simulink model "project"  (R2022a)
settings: Solver=ode45  StartTime=0.0  StopTime=100  RelTol=1e-3  EnableMultiTasking=on
libraries: simulink x2
settings Model: ExtModeTrigMode=oneshot  ExtModeArmWhenConnect=off  Creator=busvelle  LastModifiedBy=busvelle
settings SolverCC: AlgebraicLoopSolver=TrustRegion
settings DataIOCC: SaveFormat=Array  SignalLoggingSaveFormat=ModelDataLogs  ReturnWorkspaceOutputs=off
settings OptimizationCC: BlockReduction=off  BooleanDataType=off  LifeSpan=inf
settings DebuggingCC: SaveWithParameterizedLinksMsg=none  UnderspecifiedInitializationDetection=Classic  MergeDetectMultiDrivingBlocksExec=none  SignalResolutionControl=TryResolveAllWithWarning  MultiTaskDSMMsg=warning  MultiTaskCondExecSysMsg=none  UnconnectedInputMsg=warning  UnconnectedOutputMsg=warning  UnconnectedLineMsg=warning  StateNameClashWarn=warning  SFUnexpectedBacktrackingDiag=warning  SFNoUnconditionalDefaultTransitionDiag=warning  SFExecutionAtInitializationDiag=none  SFMachineParentedDataDiag=warning  ArithmeticOperatorsInVariantConditions=warning
settings HardwareCC: ProdBitPerPointer=32  ProdBitPerSizeT=32  ProdBitPerPtrDiffT=32  ProdLargestAtomicFloat=None  ProdIntDivRoundTo=Undefined  ProdEndianess=Unspecified  ProdWordSize=32  ProdHWDeviceType=32-bit Generic  TargetUnknown=on
settings ModelReferenceCC: PropagateSignalLabelsOutOfModel=off
settings SFSimCC: SimUseLocalCustomCode=off  CustomCodeUndefinedFunction=UseInterfaceOnly
settings RTWCC: RTWUseLocalCustomCode=off
settings CodeAppCC: StateflowObjectComments=on
settings GRTTargetCC: TargetLangStandard=C89/C90 (ANSI)  CombineOutputUpdateFcns=off  GRTInterface=on
settings ConfigComp: CovMetricSettings=dw  CovSaveCumulativeToWorkspaceVar=on  CovSaveSingleToWorkspaceVar=on  CovExternalEMLEnable=off

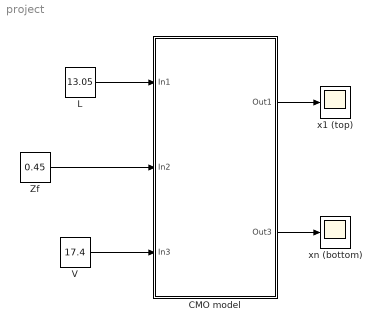
== system project ==
  CMO model : Subsystem
      mask Display: image('colonne.jpg')
  L : Constant  Value=13.05
  V : Constant  Value=17.4
  Zf : Constant  Value=0.45
  x1 (top) : Scope
  xn (bottom) : Scope
  wires:
  L/1 -> CMO model/1(In1)
  CMO model/1(Out1) -> x1 (top)/1
  V/1 -> CMO model/3(In3)
  Zf/1 -> CMO model/2(In2)
  CMO model/2(Out3) -> xn (bottom)/1

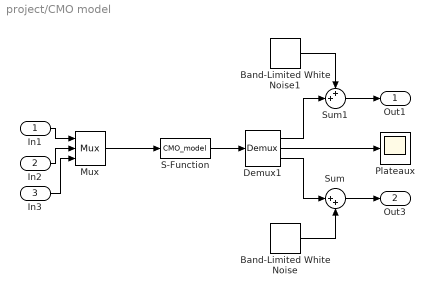
== system project/CMO model ==
  In1 : Inport
  In2 : Inport  Port=2
  In3 : Inport  Port=3
  Band-Limited White Noise : simulink/Sources/Band-Limited White Noise  Cov=[0.0001]  Ts=1  seed=[23341]
  Band-Limited White Noise1 : simulink/Sources/Band-Limited White Noise  Cov=[0.0001]  Ts=1  seed=[23341]
  Demux1 : Demux  Outputs=[1,11,1]
      settings: DisplayOption=none
  Mux : Mux  Inputs=3
  Plateaux : Scope
  S-Function : S-Function  FunctionName=CMO_model  SFunctionDeploymentMode=off  EnableBusSupport=off
  Sum : Sum  Inputs=|++
  Sum1 : Sum  Inputs=++|
  Out1 : Outport  InitialOutput=0  VectorParamsAs1DForOutWhenUnconnected=off
  Out3 : Outport  Port=2  VectorParamsAs1DForOutWhenUnconnected=off
  wires:
  In3/1 -> Mux/3
  Demux1/2 -> Plateaux/1
  S-Function/1 -> Demux1/1
  In2/1 -> Mux/2
  In1/1 -> Mux/1
  Mux/1 -> S-Function/1
  Sum/1 -> Out3/1
  Demux1/3 -> Sum/1
  Band-Limited White Noise/1 -> Sum/2
  Sum1/1 -> Out1/1
  Demux1/1 -> Sum1/2
  Band-Limited White Noise1/1 -> Sum1/1
